simulink model "mhkzq"  (R2018b)
settings: Solver=FixedStepAuto  StartTime=0.0  StopTime=1800  FixedStep=0.01  RelTol=1e-3
libraries: dspstat3 x3, fuzblock x1
settings Model: Creator=lenovo  LastModifiedBy=Allen
settings SolverCC: ZeroCrossControl=DisableAll
settings DataIOCC: LimitDataPoints=on  SaveFormat=Array
settings OptimizationCC: BlockReduction=off  BooleanDataType=off  LifeSpan=inf
settings DebuggingCC: SaveWithParameterizedLinksMsg=none  UnderspecifiedInitializationDetection=Classic  MergeDetectMultiDrivingBlocksExec=none  SignalResolutionControl=TryResolveAllWithWarning  SFUnexpectedBacktrackingDiag=warning  SFNoUnconditionalDefaultTransitionDiag=warning
settings HardwareCC: ProdBitPerPointer=32  ProdBitPerSizeT=32  ProdBitPerPtrDiffT=32  ProdLargestAtomicFloat=None  ProdIntDivRoundTo=Undefined  ProdEndianess=Unspecified  ProdWordSize=32  ProdHWDeviceType=32-bit Generic  TargetUnknown=on
settings ModelReferenceCC: PropagateSignalLabelsOutOfModel=off
settings SFSimCC: SimUseLocalCustomCode=off
settings RTWCC: RTWUseLocalCustomCode=off
settings CodeAppCC: StateflowObjectComments=on
settings GRTTargetCC: TargetLangStandard=C89/C90 (ANSI)  GeneratePreprocessorConditionals=Disable all
settings ConfigComp: CovMetricSettings=dw  CovHtmlReporting=on  CovSaveCumulativeToWorkspaceVar=on  CovSaveSingleToWorkspaceVar=on  CovExternalEMLEnable=off  CovSFcnEnable=off

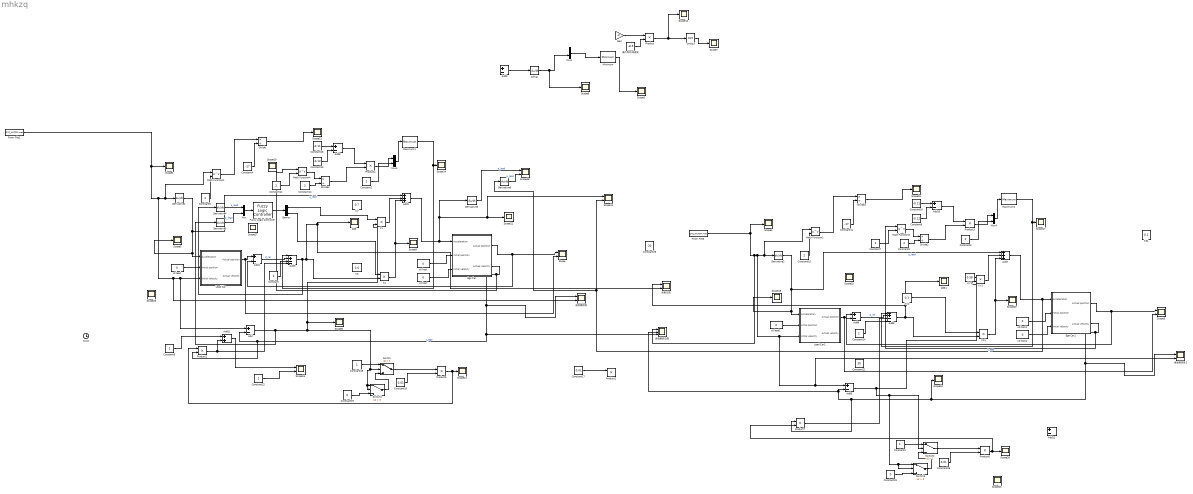
== system mhkzq ==
  Add{,2,4..6,9..10,12} (8 alike) : Sum  Inputs=+-
  Add1 : Sum  Inputs=+++
  Add11 : Sum
  Add3 : Sum  Inputs=-+--
  Add7 : Sum  Inputs=+++
  Add8 : Sum  Inputs=-+--
  Afmax : Derivative
  Clock : Clock
  Constant{,1,3,5..7,9,12,14..15,22,24} (12 alike) : Constant  Value=2
  Constant10 : Constant  Value=-0.11
  Constant11 : Constant  Value=-17
  Constant13 : Constant  Value=-0.12
  Constant16 : Constant  Value=-0.11
  Constant17 : Constant  Value=0.01
  Constant18 : Constant
  Constant19 : Constant  Value=0
  Constant2 : Constant
  Constant20 : Constant  Value=0.01
  Constant21 : Constant  Value=30
  Constant23 : Constant  Value=0
  Constant25 : Constant  Value=20
  Constant26 : Constant  Value=0.01
  Constant4 : Constant  Value=-17
  Constant8 : Constant  Value=-0.12
  Demux : Demux  Outputs=2
  Derivative{1..6} (6 alike) : Derivative
  Divide{,1..2,4} (4 alike) : Product  Inputs=*/
  Ego Car : Subsystem
  Ego Car1 : Subsystem
  From File2 : FromFile  FileName=CYC_WLTCM.mat  SampleTime=0
  From File3 : FromFile  FileName=CYC_WLTCM.mat  SampleTime=0
  Fuzzy Logic Controller : fuzblock/Fuzzy Logic  Controller  FIS='fuzzy2.fis'  OutputSampleNumber=101  DataType=double  FuzzifiedInputs=off  RuleFiringStrengths=off  RuleOutputs=off  AggregatedOutputs=off  SimulateUsing=Interpreted execution  OutOfRangeInputValueMessage=warning  NoRuleFiredMessage=warning  EmptyOutputFuzzySetMessage=warning
  Gain : Gain  Gain=-2
  KS : Constant  Value=0.6
  KS1 : Constant  Value=0.1
  KV : Constant  Value=0.7
  KV1 : Constant  Value=0.58
  KV2 : Constant  Value=0.1
  Ks : Product
  Ks1 : Product
  Kv : Product
  Kv1 : Product
  Lead Car : Subsystem
  Lead Car1 : Subsystem
  Math Function{1..4} (4 alike) : Math  Operator=pow  SaturateOnIntegerOverflow=on
  Maximum1 : dspstat3/Maximum  operation=maximum  fcn=Value  indexBase=One  operateOver=Each column  Dimension=1  InputProcessing=Columns as channels (frame based)  reset=None  roiEnable=off  roiType=Rectangles  roiPortion=Entire ROI  roiOutput=Individual statistics for each ROI  roiFlag=off  roundingMode=Floor  overflowMode=off  accumDataTypeStr=Inherit: Same as product output  accumLastDataTypeStr=Inherit: Same as product output
  Maximum2 : dspstat3/Maximum  operation=maximum  fcn=Value  indexBase=One  operateOver=Each column  Dimension=1  InputProcessing=Columns as channels (frame based)  reset=None  roiEnable=off  roiType=Rectangles  roiPortion=Entire ROI  roiOutput=Individual statistics for each ROI  roiFlag=off  roundingMode=Floor  overflowMode=off  accumDataTypeStr=Inherit: Same as product output  accumLastDataTypeStr=Inherit: Same as product output
  Minimum : dspstat3/Minimum  operation=minimum  fcn=Value  indexBase=One  operateOver=Entire input  Dimension=1  InputProcessing=Columns as channels (frame based)  reset=None  roiEnable=off  roiType=Rectangles  roiPortion=Entire ROI  roiOutput=Individual statistics for each ROI  roiFlag=off  roundingMode=Floor  overflowMode=off
      settings: SourceProductName=DSP System Toolbox  SourceProductBaseCode=DS
  Mux{,1,3..4} (4 alike) : Mux  Inputs=2
  Product{,1..7} (8 alike) : Product
  Scope{,3,11,23..25,28} (7 alike) : Scope  NumInputPorts=2
  Scope{1..2,4..10,12..22,26..27} (22 alike) : Scope
  Switch : Switch  Criteria=u2 > Threshold  Threshold=1
  Switch1 : Switch  Criteria=u2 > Threshold
  Switch2 : Switch  Criteria=u2 > Threshold  Threshold=1
  Switch3 : Switch  Criteria=u2 > Threshold
  VFMAX : Sqrt  SaturateOnIntegerOverflow=on
  v0 host : Constant  Value=0  SampleTime=0.1
  v0 host1 : Constant  Value=0  SampleTime=0.1
  x0 host : Constant  Value=0  SampleTime=0.1
  x0 host1 : Constant  Value=0  SampleTime=0.1
  x0 lead : Constant  Value=0  SampleTime=0.1
  x0 lead1 : Constant  Value=0  SampleTime=0.1
  最大制动减速度 : Constant  Value=-8.5
  误差 : Scope
  误差1 : Scope
  误差总图 : Scope  NumInputPorts=2
  速度跟踪图 : Scope  NumInputPorts=2
  速度跟踪图1 : Scope  NumInputPorts=2
  速度跟踪总图 : Scope  NumInputPorts=3
  wires:
  x0 host/1 -> Ego Car/2(Initial position)
  Derivative1/1 -> Scope5/1, Lead Car/1(Acceleration), Add1/1  "a_lead"
  x0 lead/1 -> Lead Car/2(Initial position)
  v0 host/1 -> Ego Car/3(Initial velocity)
  Ego Car/2(Actual velocity) -> Math Function4/1, 速度跟踪图/1, 速度跟踪总图/3, Product1/2, Add/2  "v_ego"
  Add/1 -> Derivative5/1, Switch1/1, Switch1/2, Switch/2, Scope8/1, Kv/2
  Kv/1 -> Add1/2
  Ks/1 -> Scope9/1, Add1/3
  Add2/1 -> Afmax/1
  Afmax/1 -> Scope6/1, Mux1/2
  Mux1/1 -> Minimum/1
  Constant/1 -> Add3/3
  Add4/1 -> Add3/2  "d_rel"
  From File2/1 -> 速度跟踪图/2, Add/1, Lead Car/3(Initial velocity), Math Function1/1, Derivative1/1, Scope1/1
  Add3/1 -> Derivative4/1, 误差总图/2, 误差/1, Ks/2
  Math Function1/1 -> Divide/1
  Constant4/1 -> Divide/2
  Divide/1 -> Scope13/1
  Gain/1 -> Product/1
  最大制动减速度/1 -> Product/2
  Product/1 -> Scope12/1, VFMAX/1
  VFMAX/1 -> Scope7/1
  Minimum/1 -> Scope2/1
  Add1/1 -> Scope11/1, Scope22/1, Derivative3/1, Ego Car/1(Acceleration)
  Ego Car/1(Actual position) -> Scope/1, Add4/2
  Lead Car/1(Actual position) -> Scope/2, Add4/1
  Constant5/1 -> Math Function1/2
  Constant12/1 -> Math Function4/2
  Product4/1 -> Mux3/1
  Constant1/1 -> Mux3/2
  Mux3/1 -> Maximum1/1
  Maximum1/1 -> Add3/1, Scope14/1
  Constant16/1 -> Add6/1
  Constant13/1 -> Add6/2
  Add6/1 -> Product4/1
  Constant14/1 -> Divide4/2
  Math Function4/1 -> Divide4/1
  Divide4/1 -> Product4/2
  Constant10/1 -> Add10/1
  Product3/1 -> Mux4/1
  Maximum2/1 -> Add8/1, Scope17/1
  Constant3/1 -> Mux4/2
  Constant8/1 -> Add10/2
  Ego Car1/2(Actual velocity) -> Math Function3/1, 速度跟踪图1/1, Scope19/1, Product7/1, 速度跟踪总图/2, Add5/2  "v_ego"
  Constant17/1 -> Product2/1
  From File3/1 -> Scope4/1, 速度跟踪总图/1, 速度跟踪图1/2, Add5/1, Lead Car1/3(Initial velocity), Math Function2/1, Derivative2/1
  Divide1/1 -> Scope16/1
  Ego Car1/1(Actual position) -> Scope3/1, Add9/2
  Add8/1 -> 误差1/1, 误差总图/1, Ks1/2
  Add5/1 -> Switch3/2, Switch3/1, Switch2/2, Kv1/2
  Add9/1 -> Add8/2  "d_rel"
  Divide2/1 -> Product3/2
  Kv1/1 -> Add7/2
  Mux4/1 -> Maximum2/1
  Derivative2/1 -> Scope18/1, Lead Car1/1(Acceleration), Add7/1  "a_lead"
  Math Function2/1 -> Divide1/1
  Add7/1 -> Scope11/2, Derivative6/1, Ego Car1/1(Acceleration)
  Ks1/1 -> Scope20/1, Add7/3
  Constant11/1 -> Divide1/2
  Lead Car1/1(Actual position) -> Scope3/2, Add9/1
  Math Function3/1 -> Divide2/1
  Add10/1 -> Product3/1
  x0 host1/1 -> Ego Car1/2(Initial position)
  v0 host1/1 -> Ego Car1/3(Initial velocity)
  Constant15/1 -> Math Function2/2
  x0 lead1/1 -> Lead Car1/2(Initial position)
  Constant9/1 -> Divide2/2
  Constant7/1 -> Math Function3/2
  Constant18/1 -> Switch/1
  Switch1/1 -> Switch/3
  Constant19/1 -> Switch1/3
  Product1/1 -> Add11/2, Add3/4
  Switch/1 -> Product5/1
  Constant20/1 -> Product5/2
  Product5/1 -> Product1/1, Scope21/1
  Constant6/1 -> Add11/1
  Add11/1 -> Scope24/1
  Constant22/1 -> Scope24/2
  Constant24/1 -> Add8/4
  Switch3/1 -> Switch2/3
  Product6/1 -> Product7/2, Scope26/1
  Constant26/1 -> Product6/2
  Switch2/1 -> Product6/1
  Constant23/1 -> Switch3/3
  Constant2/1 -> Switch2/1
  Product7/1 -> Add8/3
  KV1/1 -> Kv1/1
  KV2/1 -> Ks1/1
  Demux/1 -> Kv/1
  Demux/2 -> Ks/1
  Mux/1 -> Fuzzy Logic Controller/1
  Fuzzy Logic Controller/1 -> Demux/1
  Derivative4/1 -> Mux/1  "a_lead"
  Derivative5/1 -> Mux/2  "a_lead"
  Derivative3/1 -> Scope28/1  "a_lead"
  Derivative6/1 -> Scope28/2  "a_lead"

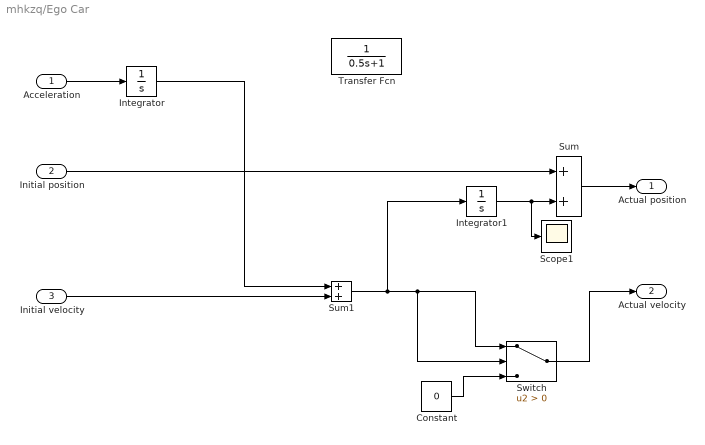
== system mhkzq/Ego Car ==
  Acceleration : Inport
  Initial position : Inport  Port=2
  Initial velocity : Inport  Port=3
  Constant : Constant  Value=0
  Integrator : Integrator
  Integrator1 : Integrator
  Scope1 : Scope
  Sum : Sum
  Sum1 : Sum
  Switch : Switch  Criteria=u2 > Threshold
  Transfer Fcn : TransferFcn  Denominator=[0.5 1]
  Actual position : Outport
  Actual velocity : Outport  Port=2
  wires:
  Initial velocity/1 -> Sum1/2
  Sum/1 -> Actual position/1
  Acceleration/1 -> Integrator/1
  Initial position/1 -> Sum/1
  Integrator1/1 -> Scope1/1, Sum/2
  Sum1/1 -> Switch/2, Switch/1, Integrator1/1
  Constant/1 -> Switch/3
  Switch/1 -> Actual velocity/1
  Integrator/1 -> Sum1/1

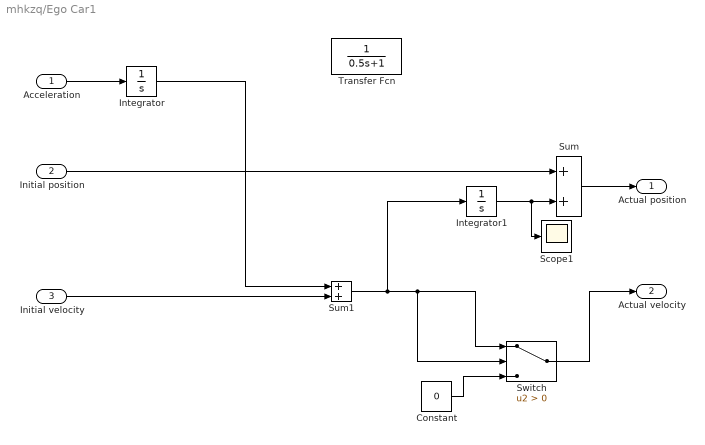
== system mhkzq/Ego Car1 ==
  Acceleration : Inport
  Initial position : Inport  Port=2
  Initial velocity : Inport  Port=3
  Constant : Constant  Value=0
  Integrator : Integrator
  Integrator1 : Integrator
  Scope1 : Scope
  Sum : Sum
  Sum1 : Sum
  Switch : Switch  Criteria=u2 > Threshold
  Transfer Fcn : TransferFcn  Denominator=[0.5 1]
  Actual position : Outport
  Actual velocity : Outport  Port=2
  wires:
  Initial velocity/1 -> Sum1/2
  Sum/1 -> Actual position/1
  Acceleration/1 -> Integrator/1
  Initial position/1 -> Sum/1
  Integrator1/1 -> Scope1/1, Sum/2
  Sum1/1 -> Switch/2, Switch/1, Integrator1/1
  Integrator/1 -> Sum1/1
  Constant/1 -> Switch/3
  Switch/1 -> Actual velocity/1

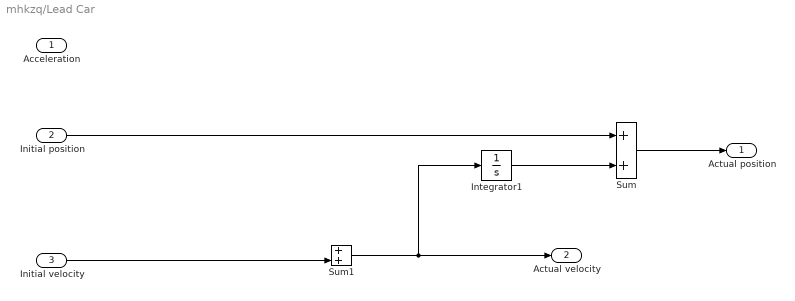
== system mhkzq/Lead Car ==
  Acceleration : Inport
  Initial position : Inport  Port=2
  Initial velocity : Inport  Port=3
  Integrator1 : Integrator
  Sum : Sum
  Sum1 : Sum
  Actual position : Outport
  Actual velocity : Outport  Port=2
  wires:
  Initial velocity/1 -> Sum1/2
  Sum/1 -> Actual position/1
  Sum1/1 -> Integrator1/1, Actual velocity/1
  Initial position/1 -> Sum/1
  Integrator1/1 -> Sum/2

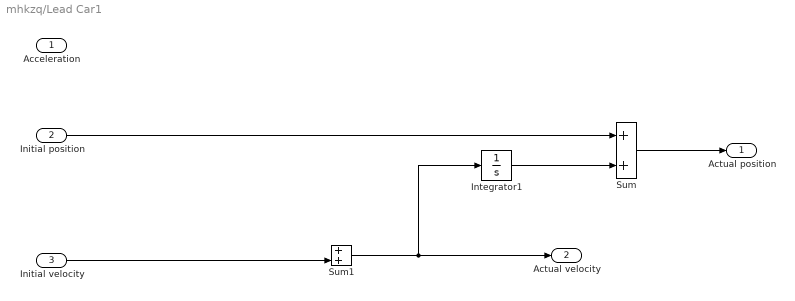
== system mhkzq/Lead Car1 ==
  Acceleration : Inport
  Initial position : Inport  Port=2
  Initial velocity : Inport  Port=3
  Integrator1 : Integrator
  Sum : Sum
  Sum1 : Sum
  Actual position : Outport
  Actual velocity : Outport  Port=2
  wires:
  Initial velocity/1 -> Sum1/2
  Sum/1 -> Actual position/1
  Sum1/1 -> Integrator1/1, Actual velocity/1
  Initial position/1 -> Sum/1
  Integrator1/1 -> Sum/2
